simulink library "hrg_wa_v10_2_cn_modules"  (R2025a)
settings: Solver=VariableStepAuto  StartTime=0.0  StopTime=10.0  RelTol=1e-3
undefined symbols (not defined in the file): Ad, Bd, p, x0
settings Model: Creator=11725  LastModifiedBy=11725

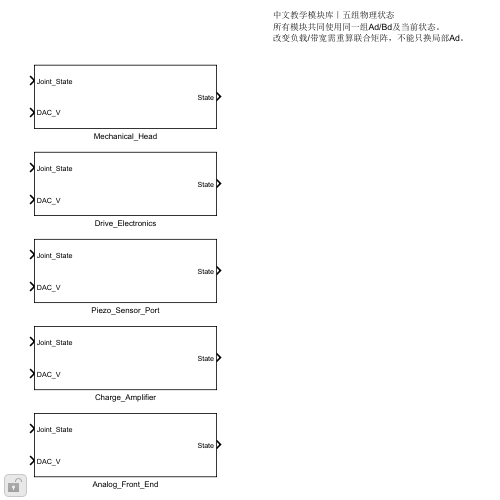
[thumbnail: Simulink's stored preview of the top-level diagram]
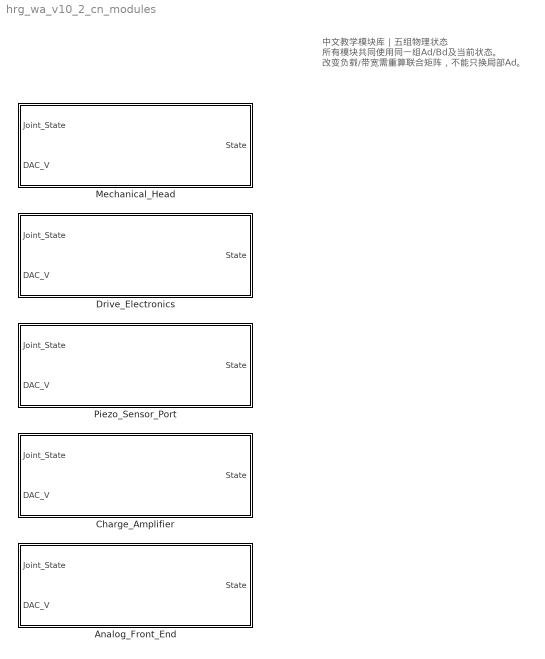
== system hrg_wa_v10_2_cn_modules ==
  note: 中文教学模块库｜五组物理状态
      | 所有模块共同使用同一组Ad/Bd及当前状态。
      | 改变负载/带宽需重算联合矩阵，不能只换局部Ad。
  Analog_Front_End : Subsystem  Description=|
      | 模拟前端AFE｜带宽及通道耦合
      | 状态11:12为ADC前电压[V]。afe_bw为Hz，内部乘2π换成角频率。
      | 检测矩阵包含两通道幅值不一致与串扰。
  Charge_Amplifier : Subsystem  Description=|
      | 电荷放大器｜积分及泄放
      | 状态9:10为输出电压[V]。Cf决定电荷/电压增益，Rf提供直流泄放。
      | 输出还需经过AFE，不能直接当作理想运动电荷。
  Drive_Electronics : Subsystem  Description=|
      | 驱动电子学｜双通道一阶带宽
      | 状态5:6为驱动器电压[V]。DAC输入为两路采样电压[V]。
      | 通道时间常数driver_tau及drive_matrix描述不一致与串扰。
  Mechanical_Head : Subsystem  Description=|
      | 机械表头｜二维二阶模态
      | 状态1:2为运动电荷r[C]，3:4为电荷速度[C/s]。
      | 刚度、阻尼可有不同主轴；角速度经科里奥利项耦合。
      | 输入是当前联合12维状态和DAC电压，不是独立机械力接口。
  Piezo_Sensor_Port : Subsystem  Description=|
      | 压电传感端口｜互易机电加载
      | 状态7:8为节点电压[V]。Cs、G0、Rs及运动电荷电流共同作用。
      | 端口电压回作用机械运动；不可把加载衰减率再次加到本征阻尼。

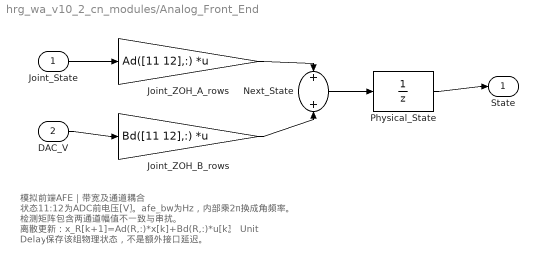
== system hrg_wa_v10_2_cn_modules/Analog_Front_End ==
  note: 模拟前端AFE｜带宽及通道耦合
      | 状态11:12为ADC前电压[V]。afe_bw为Hz，内部乘2π换成角频率。
      | 检测矩阵包含两通道幅值不一致与串扰。
      | 离散更新：x_R[k+1]=Ad(R,:)*x[k]+Bd(R,:)*u[k]。
      | Unit Delay保存该组物理状态，不是额外接口延迟。
  Joint_State : Inport
  DAC_V : Inport  Port=2
  Joint_ZOH_A_rows : Gain  Description=联合归一化ZOH的对应状态行；保留采样间隔内所有跨模块耦合。  Gain=Ad([11 12],:)  Multiplication=Matrix(K*u)
  Joint_ZOH_B_rows : Gain  Gain=Bd([11 12],:)  Multiplication=Matrix(K*u)
  Next_State : Sum
  Physical_State : UnitDelay  Description=该组唯一状态存储；初值x0(R)，采样周期p.Ts[s]。  InitialCondition=x0([11 12])  SampleTime=p.Ts  HasFrameUpgradeWarning=on
  State : Outport
  wires:
  Joint_State/1 -> Joint_ZOH_A_rows/1
  DAC_V/1 -> Joint_ZOH_B_rows/1
  Joint_ZOH_A_rows/1 -> Next_State/1
  Joint_ZOH_B_rows/1 -> Next_State/2
  Next_State/1 -> Physical_State/1
  Physical_State/1 -> State/1

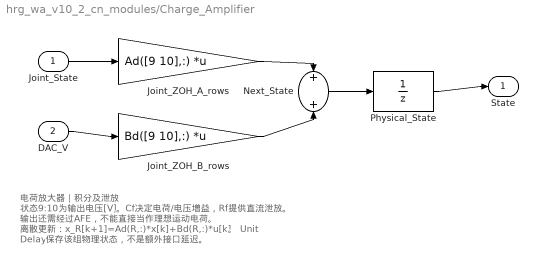
== system hrg_wa_v10_2_cn_modules/Charge_Amplifier ==
  note: 电荷放大器｜积分及泄放
      | 状态9:10为输出电压[V]。Cf决定电荷/电压增益，Rf提供直流泄放。
      | 输出还需经过AFE，不能直接当作理想运动电荷。
      | 离散更新：x_R[k+1]=Ad(R,:)*x[k]+Bd(R,:)*u[k]。
      | Unit Delay保存该组物理状态，不是额外接口延迟。
  Joint_State : Inport
  DAC_V : Inport  Port=2
  Joint_ZOH_A_rows : Gain  Description=联合归一化ZOH的对应状态行；保留采样间隔内所有跨模块耦合。  Gain=Ad([9 10],:)  Multiplication=Matrix(K*u)
  Joint_ZOH_B_rows : Gain  Gain=Bd([9 10],:)  Multiplication=Matrix(K*u)
  Next_State : Sum
  Physical_State : UnitDelay  Description=该组唯一状态存储；初值x0(R)，采样周期p.Ts[s]。  InitialCondition=x0([9 10])  SampleTime=p.Ts  HasFrameUpgradeWarning=on
  State : Outport
  wires:
  Joint_State/1 -> Joint_ZOH_A_rows/1
  DAC_V/1 -> Joint_ZOH_B_rows/1
  Joint_ZOH_A_rows/1 -> Next_State/1
  Joint_ZOH_B_rows/1 -> Next_State/2
  Next_State/1 -> Physical_State/1
  Physical_State/1 -> State/1

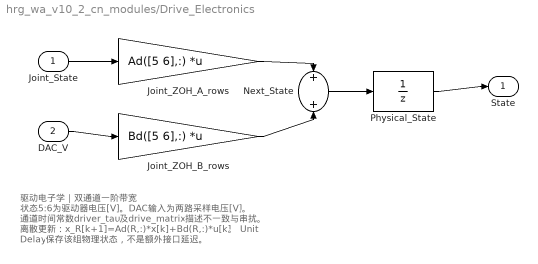
== system hrg_wa_v10_2_cn_modules/Drive_Electronics ==
  note: 驱动电子学｜双通道一阶带宽
      | 状态5:6为驱动器电压[V]。DAC输入为两路采样电压[V]。
      | 通道时间常数driver_tau及drive_matrix描述不一致与串扰。
      | 离散更新：x_R[k+1]=Ad(R,:)*x[k]+Bd(R,:)*u[k]。
      | Unit Delay保存该组物理状态，不是额外接口延迟。
  Joint_State : Inport
  DAC_V : Inport  Port=2
  Joint_ZOH_A_rows : Gain  Description=联合归一化ZOH的对应状态行；保留采样间隔内所有跨模块耦合。  Gain=Ad([5 6],:)  Multiplication=Matrix(K*u)
  Joint_ZOH_B_rows : Gain  Gain=Bd([5 6],:)  Multiplication=Matrix(K*u)
  Next_State : Sum
  Physical_State : UnitDelay  Description=该组唯一状态存储；初值x0(R)，采样周期p.Ts[s]。  InitialCondition=x0([5 6])  SampleTime=p.Ts  HasFrameUpgradeWarning=on
  State : Outport
  wires:
  Joint_State/1 -> Joint_ZOH_A_rows/1
  DAC_V/1 -> Joint_ZOH_B_rows/1
  Joint_ZOH_A_rows/1 -> Next_State/1
  Joint_ZOH_B_rows/1 -> Next_State/2
  Next_State/1 -> Physical_State/1
  Physical_State/1 -> State/1

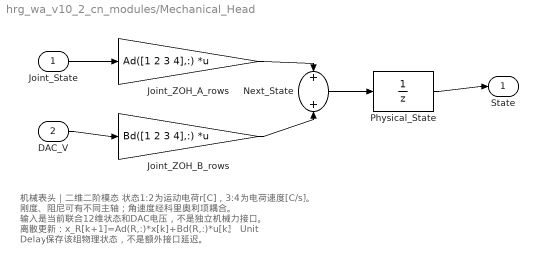
== system hrg_wa_v10_2_cn_modules/Mechanical_Head ==
  note: 机械表头｜二维二阶模态
      | 状态1:2为运动电荷r[C]，3:4为电荷速度[C/s]。
      | 刚度、阻尼可有不同主轴；角速度经科里奥利项耦合。
      | 输入是当前联合12维状态和DAC电压，不是独立机械力接口。
      | 离散更新：x_R[k+1]=Ad(R,:)*x[k]+Bd(R,:)*u[k]。
      | Unit Delay保存该组物理状态，不是额外接口延迟。
  Joint_State : Inport
  DAC_V : Inport  Port=2
  Joint_ZOH_A_rows : Gain  Description=联合归一化ZOH的对应状态行；保留采样间隔内所有跨模块耦合。  Gain=Ad([1 2 3 4],:)  Multiplication=Matrix(K*u)
  Joint_ZOH_B_rows : Gain  Gain=Bd([1 2 3 4],:)  Multiplication=Matrix(K*u)
  Next_State : Sum
  Physical_State : UnitDelay  Description=该组唯一状态存储；初值x0(R)，采样周期p.Ts[s]。  InitialCondition=x0([1 2 3 4])  SampleTime=p.Ts  HasFrameUpgradeWarning=on
  State : Outport
  wires:
  Joint_State/1 -> Joint_ZOH_A_rows/1
  DAC_V/1 -> Joint_ZOH_B_rows/1
  Joint_ZOH_A_rows/1 -> Next_State/1
  Joint_ZOH_B_rows/1 -> Next_State/2
  Next_State/1 -> Physical_State/1
  Physical_State/1 -> State/1

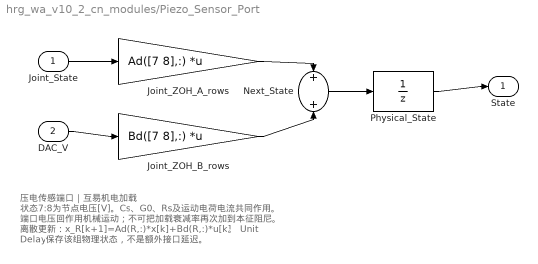
== system hrg_wa_v10_2_cn_modules/Piezo_Sensor_Port ==
  note: 压电传感端口｜互易机电加载
      | 状态7:8为节点电压[V]。Cs、G0、Rs及运动电荷电流共同作用。
      | 端口电压回作用机械运动；不可把加载衰减率再次加到本征阻尼。
      | 离散更新：x_R[k+1]=Ad(R,:)*x[k]+Bd(R,:)*u[k]。
      | Unit Delay保存该组物理状态，不是额外接口延迟。
  Joint_State : Inport
  DAC_V : Inport  Port=2
  Joint_ZOH_A_rows : Gain  Description=联合归一化ZOH的对应状态行；保留采样间隔内所有跨模块耦合。  Gain=Ad([7 8],:)  Multiplication=Matrix(K*u)
  Joint_ZOH_B_rows : Gain  Gain=Bd([7 8],:)  Multiplication=Matrix(K*u)
  Next_State : Sum
  Physical_State : UnitDelay  Description=该组唯一状态存储；初值x0(R)，采样周期p.Ts[s]。  InitialCondition=x0([7 8])  SampleTime=p.Ts  HasFrameUpgradeWarning=on
  State : Outport
  wires:
  Joint_State/1 -> Joint_ZOH_A_rows/1
  DAC_V/1 -> Joint_ZOH_B_rows/1
  Joint_ZOH_A_rows/1 -> Next_State/1
  Joint_ZOH_B_rows/1 -> Next_State/2
  Next_State/1 -> Physical_State/1
  Physical_State/1 -> State/1
